simulink model "dairy_cip_digital_twin_publication_clean"  (R2026a)
settings: Solver=ode23t  StopTime=1900  MaxStep=5  RelTol=1e-4
PostLoadFcn:
  | try
  |     model_name = 'dairy_cip_digital_twin';
  |     model_file = get_param(model_name, 'FileName');
  |     if ~isempty(model_file)
  |         project_root = fileparts(fileparts(model_file));
  |     else
  |         project_root = pwd;
  |     end
  |     src_dir = fullfile(project_root, 'src');
  |     if ~isfolder(src_dir)
  |         src_dir = fullfile(pwd, 'src');
  |     end
  |     if isfolder(src_dir)
  |         addpath(src_dir);
  |     end
  | catch ME
  |     warning('dairy_cip_digital_twin:pathSetupFailed', ...
  |         'Could not add project src to MATLAB path: %s', ME.message);
  | end
InitFcn:
  | try
  |     model_name = 'dairy_cip_digital_twin';
  |     model_file = get_param(model_name, 'FileName');
  |     if ~isempty(model_file)
  |         project_root = fileparts(fileparts(model_file));
  |     else
  |         project_root = pwd;
  |     end
  |     src_dir = fullfile(project_root, 'src');
  |     if ~isfolder(src_dir)
  |         src_dir = fullfile(pwd, 'src');
  |     end
  |     if isfolder(src_dir)
  |         addpath(src_dir);
  |     end
  | catch ME
  |     warning('dairy_cip_digital_twin:pathSetupFailed', ...
  |         'Could not add project src to MATLAB path: %s', ME.message);
  | end
model workspace (MAT data in the model file):
  NaOH_pct = 1.5
  Q_m3h = 1.5
  T_C = 65
  T_in_C = 15
  heat_rec = 0.3
  soil0 = 0.6
  t_alk = 900
  t_final = 400
  t_int = 300
  t_pre = 300
  water_rec = 0.2
settings Model: Creator=OK  LastModifiedBy=OK

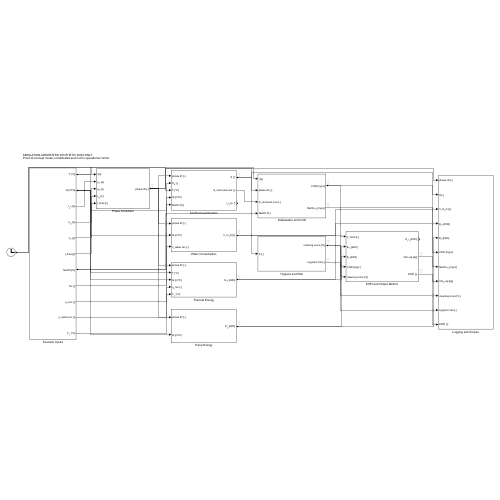
[thumbnail: Simulink's stored preview of the top-level diagram]
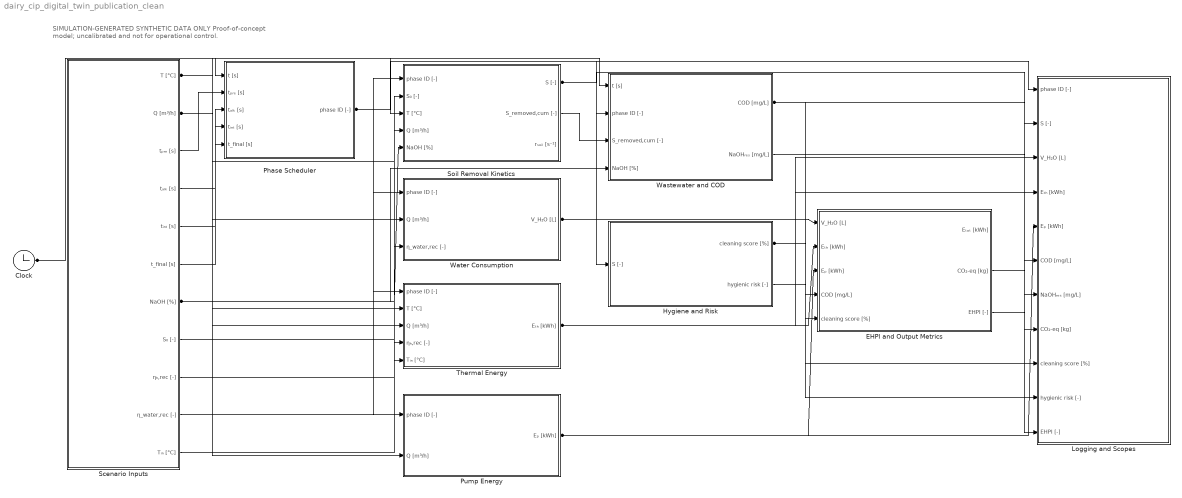
== system dairy_cip_digital_twin_publication_clean ==
  note: SIMULATION-GENERATED SYNTHETIC DATA ONLY
      | Proof-of-concept model; uncalibrated and not for operational control.
  Clock : Clock
  EHPI and Output Metrics : Subsystem
  Hygiene and Risk : Subsystem
  Logging and Scopes : Subsystem
  Phase Scheduler : Subsystem
  Pump Energy : Subsystem
  Scenario Inputs : Subsystem
  Soil Removal Kinetics : Subsystem
  Thermal Energy : Subsystem
  Wastewater and COD : Subsystem
  Water Consumption : Subsystem
  wires:
  Clock/1 -> Phase Scheduler/1(t [s]), Wastewater and COD/1(t [s])
  Scenario Inputs/3(tₚᵣₑ [s]) -> Phase Scheduler/2(tₚᵣₑ [s])
  Scenario Inputs/4(tₐₗₖ [s]) -> Phase Scheduler/3(tₐₗₖ [s])
  Scenario Inputs/5(tᵢₙₜ [s]) -> Phase Scheduler/4(tᵢₙₜ [s])
  Scenario Inputs/6(t_final [s]) -> Phase Scheduler/5(t_final [s])
  Phase Scheduler/1(phase ID [-]) -> Soil Removal Kinetics/1(phase ID [-]), Water Consumption/1(phase ID [-]), Thermal Energy/1(phase ID [-]), Pump Energy/1(phase ID [-]), Wastewater and COD/2(phase ID [-]), Logging and Scopes/1(phase ID [-])
  Scenario Inputs/8(S₀ [-]) -> Soil Removal Kinetics/2(S₀ [-])
  Scenario Inputs/1(T [°C]) -> Soil Removal Kinetics/3(T [°C]), Thermal Energy/2(T [°C])
  Scenario Inputs/2(Q [m³/h]) -> Soil Removal Kinetics/4(Q [m³/h]), Water Consumption/2(Q [m³/h]), Thermal Energy/3(Q [m³/h]), Pump Energy/2(Q [m³/h])
  Scenario Inputs/7(NaOH [%]) -> Soil Removal Kinetics/5(NaOH [%]), Wastewater and COD/4(NaOH [%])
  Scenario Inputs/10(η_water,rec [-]) -> Water Consumption/3(η_water,rec [-])
  Scenario Inputs/9(ηₕ,rec [-]) -> Thermal Energy/4(ηₕ,rec [-])
  Scenario Inputs/11(Tᵢₙ [°C]) -> Thermal Energy/5(Tᵢₙ [°C])
  Soil Removal Kinetics/2(S_removed,cum [-]) -> Wastewater and COD/3(S_removed,cum [-])
  Soil Removal Kinetics/1(S [-]) -> Hygiene and Risk/1(S [-]), Logging and Scopes/2(S [-])
  Water Consumption/1(V_H₂O [L]) -> EHPI and Output Metrics/1(V_H₂O [L]), Logging and Scopes/3(V_H₂O [L])
  Thermal Energy/1(Eₜₕ [kWh]) -> EHPI and Output Metrics/2(Eₜₕ [kWh]), Logging and Scopes/4(Eₜₕ [kWh])
  Pump Energy/1(Eₚ [kWh]) -> EHPI and Output Metrics/3(Eₚ [kWh]), Logging and Scopes/5(Eₚ [kWh])
  Wastewater and COD/1(COD [mg/L]) -> EHPI and Output Metrics/4(COD [mg/L]), Logging and Scopes/6(COD [mg/L])
  Hygiene and Risk/1(cleaning score [%]) -> EHPI and Output Metrics/5(cleaning score [%]), Logging and Scopes/9(cleaning score [%])
  Wastewater and COD/2(NaOHᵣₑₛ [mg/L]) -> Logging and Scopes/7(NaOHᵣₑₛ [mg/L])
  EHPI and Output Metrics/2(CO₂-eq [kg]) -> Logging and Scopes/8(CO₂-eq [kg])
  Hygiene and Risk/2(hygienic risk [-]) -> Logging and Scopes/10(hygienic risk [-])
  EHPI and Output Metrics/3(EHPI [-]) -> Logging and Scopes/11(EHPI [-])

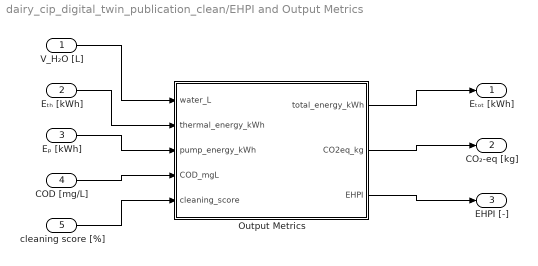
== system dairy_cip_digital_twin_publication_clean/EHPI and Output Metrics ==
  V_H₂O [L] : Inport
  Eₜₕ [kWh] : Inport  Port=2
  Eₚ [kWh] : Inport  Port=3
  COD [mg/L] : Inport  Port=4
  cleaning score [%] : Inport  Port=5
  Output Metrics : MATLAB Function  TreatAsAtomicUnit=on
  Eₜₒₜ [kWh] : Outport
  CO₂-eq [kg] : Outport  Port=2
  EHPI [-] : Outport  Port=3
  wires:
  V_H₂O [L]/1 -> Output Metrics/1(water_L)
  Eₜₕ [kWh]/1 -> Output Metrics/2(thermal_energy_kWh)
  Eₚ [kWh]/1 -> Output Metrics/3(pump_energy_kWh)
  COD [mg/L]/1 -> Output Metrics/4(COD_mgL)
  cleaning score [%]/1 -> Output Metrics/5(cleaning_score)
  Output Metrics/1(total_energy_kWh) -> Eₜₒₜ [kWh]/1
  Output Metrics/2(CO2eq_kg) -> CO₂-eq [kg]/1
  Output Metrics/3(EHPI) -> EHPI [-]/1

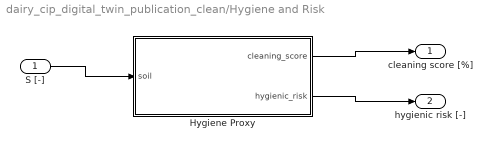
== system dairy_cip_digital_twin_publication_clean/Hygiene and Risk ==
  S [-] : Inport
  Hygiene Proxy : MATLAB Function  TreatAsAtomicUnit=on
  cleaning score [%] : Outport
  hygienic risk [-] : Outport  Port=2
  wires:
  S [-]/1 -> Hygiene Proxy/1(soil)
  Hygiene Proxy/1(cleaning_score) -> cleaning score [%]/1
  Hygiene Proxy/2(hygienic_risk) -> hygienic risk [-]/1

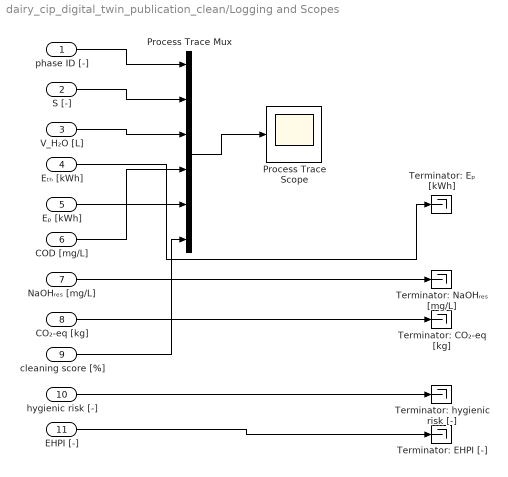
== system dairy_cip_digital_twin_publication_clean/Logging and Scopes ==
  phase ID [-] : Inport
  S [-] : Inport  Port=2
  V_H₂O [L] : Inport  Port=3
  Eₜₕ [kWh] : Inport  Port=4
  Eₚ [kWh] : Inport  Port=5
  COD [mg/L] : Inport  Port=6
  NaOHᵣₑₛ [mg/L] : Inport  Port=7
  CO₂-eq [kg] : Inport  Port=8
  cleaning score [%] : Inport  Port=9
  hygienic risk [-] : Inport  Port=10
  EHPI [-] : Inport  Port=11
  Process Trace Mux : Mux  Inputs=6
  Process Trace Scope : Scope
  Terminator: CO₂-eq [kg] : Terminator
  Terminator: EHPI [-] : Terminator
  Terminator: Eₚ [kWh] : Terminator
  Terminator: NaOHᵣₑₛ [mg/L] : Terminator
  Terminator: hygienic risk [-] : Terminator
  wires:
  phase ID [-]/1 -> Process Trace Mux/1
  S [-]/1 -> Process Trace Mux/2
  V_H₂O [L]/1 -> Process Trace Mux/3
  COD [mg/L]/1 -> Process Trace Mux/4
  Eₜₕ [kWh]/1 -> Process Trace Mux/5
  cleaning score [%]/1 -> Process Trace Mux/6
  Process Trace Mux/1 -> Process Trace Scope/1
  Eₚ [kWh]/1 -> Terminator: Eₚ [kWh]/1
  NaOHᵣₑₛ [mg/L]/1 -> Terminator: NaOHᵣₑₛ [mg/L]/1
  CO₂-eq [kg]/1 -> Terminator: CO₂-eq [kg]/1
  hygienic risk [-]/1 -> Terminator: hygienic risk [-]/1
  EHPI [-]/1 -> Terminator: EHPI [-]/1

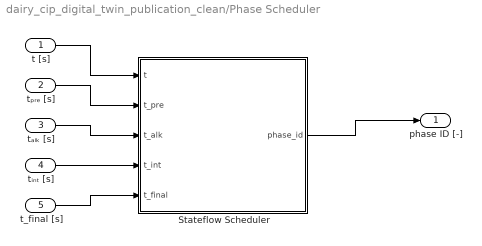
== system dairy_cip_digital_twin_publication_clean/Phase Scheduler ==
  t [s] : Inport
  tₚᵣₑ [s] : Inport  Port=2
  tₐₗₖ [s] : Inport  Port=3
  tᵢₙₜ [s] : Inport  Port=4
  t_final [s] : Inport  Port=5
  Stateflow Scheduler : Stateflow chart  TreatAsAtomicUnit=on
  phase ID [-] : Outport
  wires:
  t [s]/1 -> Stateflow Scheduler/1(t)
  tₚᵣₑ [s]/1 -> Stateflow Scheduler/2(t_pre)
  tₐₗₖ [s]/1 -> Stateflow Scheduler/3(t_alk)
  tᵢₙₜ [s]/1 -> Stateflow Scheduler/4(t_int)
  t_final [s]/1 -> Stateflow Scheduler/5(t_final)
  Stateflow Scheduler/1(phase_id) -> phase ID [-]/1

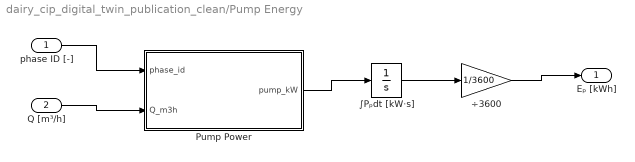
== system dairy_cip_digital_twin_publication_clean/Pump Energy ==
  phase ID [-] : Inport
  Q [m³/h] : Inport  Port=2
  Pump Power : MATLAB Function  TreatAsAtomicUnit=on
  ÷3600 : Gain  Gain=1/3600
  ∫Pₚdt [kW·s] : Integrator
  Eₚ [kWh] : Outport
  wires:
  phase ID [-]/1 -> Pump Power/1(phase_id)
  Q [m³/h]/1 -> Pump Power/2(Q_m3h)
  Pump Power/1(pump_kW) -> ∫Pₚdt [kW·s]/1
  ∫Pₚdt [kW·s]/1 -> ÷3600/1
  ÷3600/1 -> Eₚ [kWh]/1

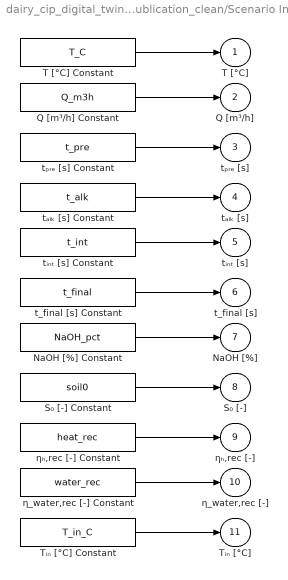
== system dairy_cip_digital_twin_publication_clean/Scenario Inputs ==
  NaOH [%] Constant : Constant  Value=NaOH_pct
  Q [m³/h] Constant : Constant  Value=Q_m3h
  S₀ [-] Constant : Constant  Value=soil0
  T [°C] Constant : Constant  Value=T_C
  Tᵢₙ [°C] Constant : Constant  Value=T_in_C
  t_final [s] Constant : Constant  Value=t_final
  tᵢₙₜ [s] Constant : Constant  Value=t_int
  tₐₗₖ [s] Constant : Constant  Value=t_alk
  tₚᵣₑ [s] Constant : Constant  Value=t_pre
  η_water,rec [-] Constant : Constant  Value=water_rec
  ηₕ,rec [-] Constant : Constant  Value=heat_rec
  T [°C] : Outport
  Q [m³/h] : Outport  Port=2
  tₚᵣₑ [s] : Outport  Port=3
  tₐₗₖ [s] : Outport  Port=4
  tᵢₙₜ [s] : Outport  Port=5
  t_final [s] : Outport  Port=6
  NaOH [%] : Outport  Port=7
  S₀ [-] : Outport  Port=8
  ηₕ,rec [-] : Outport  Port=9
  η_water,rec [-] : Outport  Port=10
  Tᵢₙ [°C] : Outport  Port=11
  wires:
  T [°C] Constant/1 -> T [°C]/1
  Q [m³/h] Constant/1 -> Q [m³/h]/1
  tₚᵣₑ [s] Constant/1 -> tₚᵣₑ [s]/1
  tₐₗₖ [s] Constant/1 -> tₐₗₖ [s]/1
  tᵢₙₜ [s] Constant/1 -> tᵢₙₜ [s]/1
  t_final [s] Constant/1 -> t_final [s]/1
  NaOH [%] Constant/1 -> NaOH [%]/1
  S₀ [-] Constant/1 -> S₀ [-]/1
  ηₕ,rec [-] Constant/1 -> ηₕ,rec [-]/1
  η_water,rec [-] Constant/1 -> η_water,rec [-]/1
  Tᵢₙ [°C] Constant/1 -> Tᵢₙ [°C]/1

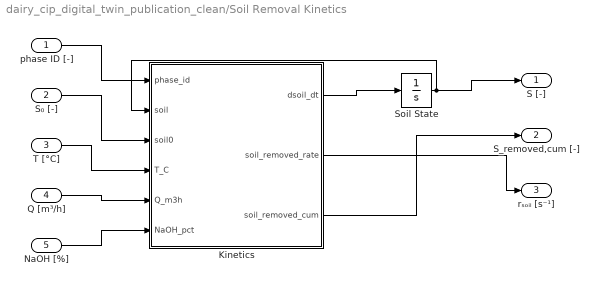
== system dairy_cip_digital_twin_publication_clean/Soil Removal Kinetics ==
  phase ID [-] : Inport
  S₀ [-] : Inport  Port=2
  T [°C] : Inport  Port=3
  Q [m³/h] : Inport  Port=4
  NaOH [%] : Inport  Port=5
  Kinetics : MATLAB Function  TreatAsAtomicUnit=on
  Soil State : Integrator  InitialCondition=soil0
  S [-] : Outport
  S_removed,cum [-] : Outport  Port=2
  rₛₒᵢₗ [s⁻¹] : Outport  Port=3
  wires:
  phase ID [-]/1 -> Kinetics/1(phase_id)
  Soil State/1 -> Kinetics/2(soil), S [-]/1
  S₀ [-]/1 -> Kinetics/3(soil0)
  T [°C]/1 -> Kinetics/4(T_C)
  Q [m³/h]/1 -> Kinetics/5(Q_m3h)
  NaOH [%]/1 -> Kinetics/6(NaOH_pct)
  Kinetics/1(dsoil_dt) -> Soil State/1
  Kinetics/3(soil_removed_cum) -> S_removed,cum [-]/1
  Kinetics/2(soil_removed_rate) -> rₛₒᵢₗ [s⁻¹]/1

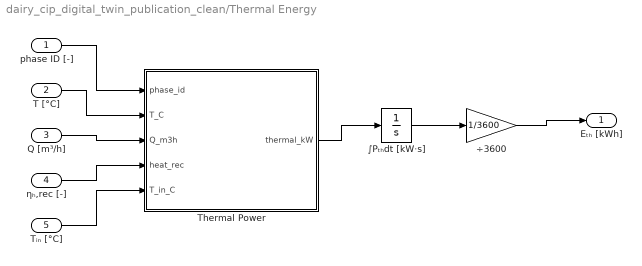
== system dairy_cip_digital_twin_publication_clean/Thermal Energy ==
  phase ID [-] : Inport
  T [°C] : Inport  Port=2
  Q [m³/h] : Inport  Port=3
  ηₕ,rec [-] : Inport  Port=4
  Tᵢₙ [°C] : Inport  Port=5
  Thermal Power : MATLAB Function  TreatAsAtomicUnit=on
  ÷3600 : Gain  Gain=1/3600
  ∫Pₜₕdt [kW·s] : Integrator
  Eₜₕ [kWh] : Outport
  wires:
  phase ID [-]/1 -> Thermal Power/1(phase_id)
  T [°C]/1 -> Thermal Power/2(T_C)
  Q [m³/h]/1 -> Thermal Power/3(Q_m3h)
  ηₕ,rec [-]/1 -> Thermal Power/4(heat_rec)
  Tᵢₙ [°C]/1 -> Thermal Power/5(T_in_C)
  Thermal Power/1(thermal_kW) -> ∫Pₜₕdt [kW·s]/1
  ∫Pₜₕdt [kW·s]/1 -> ÷3600/1
  ÷3600/1 -> Eₜₕ [kWh]/1

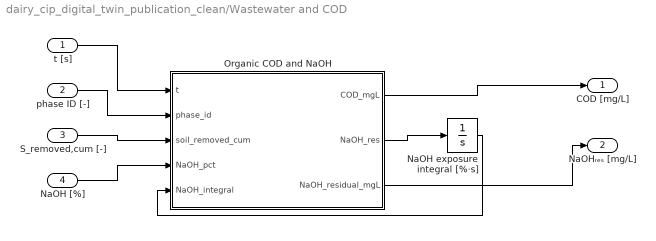
== system dairy_cip_digital_twin_publication_clean/Wastewater and COD ==
  t [s] : Inport
  phase ID [-] : Inport  Port=2
  S_removed,cum [-] : Inport  Port=3
  NaOH [%] : Inport  Port=4
  NaOH exposure integral [%·s] : Integrator
  Organic COD and NaOH : MATLAB Function  TreatAsAtomicUnit=on
  COD [mg/L] : Outport
  NaOHᵣₑₛ [mg/L] : Outport  Port=2
  wires:
  t [s]/1 -> Organic COD and NaOH/1(t)
  phase ID [-]/1 -> Organic COD and NaOH/2(phase_id)
  S_removed,cum [-]/1 -> Organic COD and NaOH/3(soil_removed_cum)
  NaOH [%]/1 -> Organic COD and NaOH/4(NaOH_pct)
  NaOH exposure integral [%·s]/1 -> Organic COD and NaOH/5(NaOH_integral)
  Organic COD and NaOH/1(COD_mgL) -> COD [mg/L]/1
  Organic COD and NaOH/2(NaOH_res) -> NaOH exposure integral [%·s]/1
  Organic COD and NaOH/3(NaOH_residual_mgL) -> NaOHᵣₑₛ [mg/L]/1

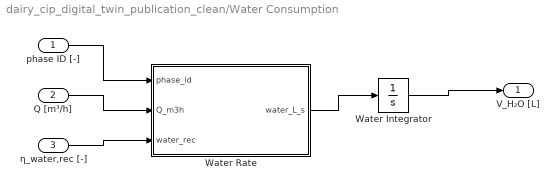
== system dairy_cip_digital_twin_publication_clean/Water Consumption ==
  phase ID [-] : Inport
  Q [m³/h] : Inport  Port=2
  η_water,rec [-] : Inport  Port=3
  Water Integrator : Integrator
  Water Rate : MATLAB Function  TreatAsAtomicUnit=on
  V_H₂O [L] : Outport
  wires:
  phase ID [-]/1 -> Water Rate/1(phase_id)
  Q [m³/h]/1 -> Water Rate/2(Q_m3h)
  η_water,rec [-]/1 -> Water Rate/3(water_rec)
  Water Rate/1(water_L_s) -> Water Integrator/1
  Water Integrator/1 -> V_H₂O [L]/1

== matlab function dairy_cip_digital_twin_publication_clean/Water Consumption/Water Rate ==
  data: phase_id input; water_L_s output; Q_m3h input; water_rec input
function water_L_s = water_rate(phase_id, Q_m3h, water_rec) %#codegen
%WATER_RATE Fresh-water flow during active CIP phases.
if phase_id >= 1 && phase_id <= 4
    water_L_s = Q_m3h * 1000 / 3600 * (1 - water_rec);
else
    water_L_s = 0;
end
end

== matlab function dairy_cip_digital_twin_publication_clean/Soil Removal Kinetics/Kinetics ==
  data: phase_id input; dsoil_dt output; soil input; soil0 input; T_C input; Q_m3h input; NaOH_pct input; soil_removed_rate output; soil_removed_cum output
function [dsoil_dt, soil_removed_rate, soil_removed_cum] = kinetics(phase_id, soil, soil0, T_C, Q_m3h, NaOH_pct) %#codegen
%KINETICS First-order soil removal for synthetic dairy CIP.
M = cip_model_params();
soil_c = max(soil, 0);
if phase_id == 1
    k = M.k_cal * M.k_pre_base * (Q_m3h / M.Q_ref)^M.beta_Q;
elseif phase_id == 2
    k = M.k_cal * M.k_alk_base * exp(M.alpha_T*(T_C - M.T_ref)) * ...
        (Q_m3h / M.Q_ref)^M.beta_Q * (NaOH_pct / M.NaOH_ref)^M.gamma_NaOH;
elseif phase_id == 3 || phase_id == 4
    k = M.k_cal * M.k_rinse_base * (Q_m3h / M.Q_ref)^M.beta_Q;
else
    k = 0;
end
dsoil_dt = -k * soil_c;
soil_removed_rate = max(-dsoil_dt, 0);
soil_removed_cum = min(max(soil0 - soil_c, 0), max(soil0, 0));
end

== stateflow chart dairy_cip_digital_twin_publication_clean/Phase Scheduler/Stateflow Scheduler ==
  state PRE_RINSE
    entry: phase_id = 1;
  state ALKALINE_WASH
    entry: phase_id = 2;
  state INTERMEDIATE_RINSE
    entry: phase_id = 3;
  state FINAL_RINSE
    entry: phase_id = 4;
  state ENDING
    entry: phase_id = 5;
  (default) -> PRE_RINSE
  PRE_RINSE -> ALKALINE_WASH : [t > t_pre]
  ALKALINE_WASH -> INTERMEDIATE_RINSE : [t > t_pre + t_alk]
  INTERMEDIATE_RINSE -> FINAL_RINSE : [t > t_pre + t_alk + t_int]
  FINAL_RINSE -> ENDING : [t > t_pre + t_alk + t_int + t_final]
  data: t input; t_pre input; t_alk input; t_int input; t_final input; phase_id output

== matlab function dairy_cip_digital_twin_publication_clean/Thermal Energy/Thermal Power ==
  data: phase_id input; thermal_kW output; T_C input; Q_m3h input; heat_rec input; T_in_C input
function thermal_kW = thermal_power(phase_id, T_C, Q_m3h, heat_rec, T_in_C) %#codegen
%THERMAL_POWER Heating power for the alkaline wash phase.
M = cip_model_params();
if phase_id == 2
    Q_m3s = Q_m3h / 3600;
    m_dot = M.rho * Q_m3s;
    dTemp = max(T_C - T_in_C, 0);
    thermal_kW = m_dot * M.cp * dTemp / M.eta_heater * (1 - heat_rec);
else
    thermal_kW = 0;
end
end

== matlab function dairy_cip_digital_twin_publication_clean/Pump Energy/Pump Power ==
  data: phase_id input; pump_kW output; Q_m3h input
function pump_kW = pump_power(phase_id, Q_m3h) %#codegen
%PUMP_POWER Pumping power during active CIP phases.
M = cip_model_params();
if phase_id >= 1 && phase_id <= 4
    Q_m3s = Q_m3h / 3600;
    pump_kW = (M.deltaP * Q_m3s / M.eta_pump) / 1000;
else
    pump_kW = 0;
end
end

== matlab function dairy_cip_digital_twin_publication_clean/Wastewater and COD/Organic COD and NaOH ==
  data: t input; COD_mgL output; phase_id input; soil_removed_cum input; NaOH_pct input; NaOH_integral input; NaOH_res output; NaOH_residual_mgL output
function [COD_mgL, NaOH_res, NaOH_residual_mgL] = wastewater_cod(t, phase_id, soil_removed_cum, NaOH_pct, NaOH_integral) %#codegen
%WASTEWATER_COD Organic COD proxy and separate NaOH residual reporting.
M = cip_model_params();
COD_mgL = M.COD_factor * max(soil_removed_cum, 0);
if phase_id == 2
    NaOH_res = NaOH_pct * 10000;
elseif phase_id == 3
    NaOH_res = NaOH_pct * 1500;
elseif phase_id == 4
    NaOH_res = NaOH_pct * 300;
else
    NaOH_res = 0;
end
NaOH_residual_mgL = NaOH_integral / max(t, M.eps_time);
end

== matlab function dairy_cip_digital_twin_publication_clean/Hygiene and Risk/Hygiene Proxy ==
  data: soil input; cleaning_score output; hygienic_risk output
function [cleaning_score, hygienic_risk] = hygiene_proxy(soil) %#codegen
%HYGIENE_PROXY Residual-soil hygiene proxies for synthetic data.
M = cip_model_params();
soil_c = max(soil, 0);
cleaning_score = max(0, min(100, (1 - soil_c) * 100));
hygienic_risk = max(0, min(1, soil_c / M.soil_risk_ref));
end

== matlab function dairy_cip_digital_twin_publication_clean/EHPI and Output Metrics/Output Metrics ==
  data: water_L input; total_energy_kWh output; thermal_energy_kWh input; pump_energy_kWh input; COD_mgL input; cleaning_score input; CO2eq_kg output; EHPI output
function [total_energy_kWh, CO2eq_kg, EHPI] = output_metrics(water_L, thermal_energy_kWh, pump_energy_kWh, COD_mgL, cleaning_score) %#codegen
%OUTPUT_METRICS Derived synthetic environmental and hygiene metrics.
M = cip_model_params();
total_energy_kWh = thermal_energy_kWh + pump_energy_kWh;
CO2eq_kg = thermal_energy_kWh * M.EF_thermal + pump_energy_kWh * M.EF_electricity;
water_norm = water_L / M.norm_water_L;
energy_norm = total_energy_kWh / M.norm_energy_kWh;
COD_norm = COD_mgL / M.norm_COD_mgL;
CO2_norm = CO2eq_kg / M.norm_CO2eq_kg;
cleaning_norm = cleaning_score / 100;
penalty_env = 0.25*water_norm + 0.25*energy_norm + 0.25*COD_norm + 0.25*CO2_norm;
EHPI = 100 * cleaning_norm / (1 + penalty_env);
end
